simulink model "simulink_scheme_task2"  (R2023b)
settings: Solver=ode4  StartTime=0.0  StopTime=simulationParameters.T_sim  FixedStep=simulationParameters.T_integration  RelTol=1e-3
values from neighbouring files (symbols this model uses):
  patientParameters = loadPatientParameter(patientID)    [main_task_2.m]
  simulationParameters = loadSimulationParameter    [main_task_2.m]
settings Model: Creator=william  LastModifiedBy=william
settings DataIOCC: ReturnWorkspaceOutputs=off
settings ConfigComp: CovBoundaryAbsTol=1.0e-5

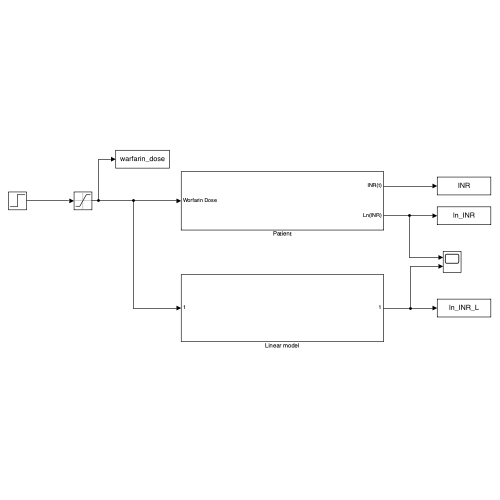
[thumbnail: Simulink's stored preview of the top-level diagram]
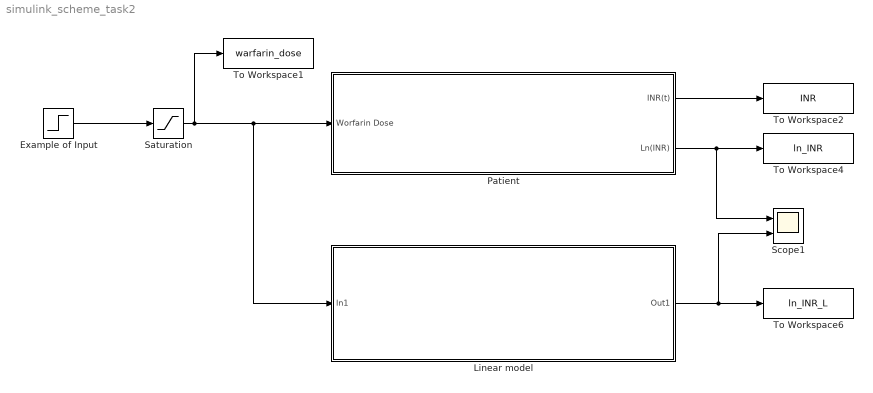
== system simulink_scheme_task2 ==
  Example of Input : Step  Time=48  After=4  SampleTime=simulationParameters.Ts
  Linear model : Subsystem
  Patient : Subsystem
  Saturation : Saturate  UpperLimit=simulationParameters.u_max  LowerLimit=simulationParameters.u_min
  Scope1 : Scope  NumInputPorts=2
  To Workspace1 : ToWorkspace  VariableName=warfarin_dose  SaveFormat=Structure With Time  SampleTime=-1
  To Workspace2 : ToWorkspace  VariableName=INR  SaveFormat=Structure With Time  SampleTime=-1
  To Workspace4 : ToWorkspace  VariableName=ln_INR  SaveFormat=Structure With Time  SampleTime=-1
  To Workspace6 : ToWorkspace  VariableName=ln_INR_L  SaveFormat=Structure With Time  SampleTime=-1
  wires:
  Saturation/1 -> Linear model/1(In1), Patient/1(Worfarin Dose), To Workspace1/1
  Patient/1(INR(t)) -> To Workspace2/1
  Patient/2(Ln(INR)) -> To Workspace4/1, Scope1/1
  Linear model/1(Out1) -> To Workspace6/1, Scope1/2
  Example of Input/1 -> Saturation/1

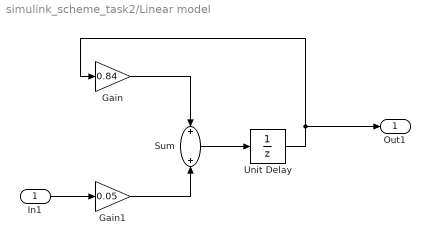
== system simulink_scheme_task2/Linear model ==
  In1 : Inport
  Gain : Gain  Gain=0.84
  Gain1 : Gain  Gain=0.05
  Sum : Sum
  Unit Delay : UnitDelay  SampleTime=simulationParameters.Ts
  Out1 : Outport
  wires:
  In1/1 -> Gain1/1
  Gain1/1 -> Sum/2
  Unit Delay/1 -> Gain/1, Out1/1
  Gain/1 -> Sum/1
  Sum/1 -> Unit Delay/1

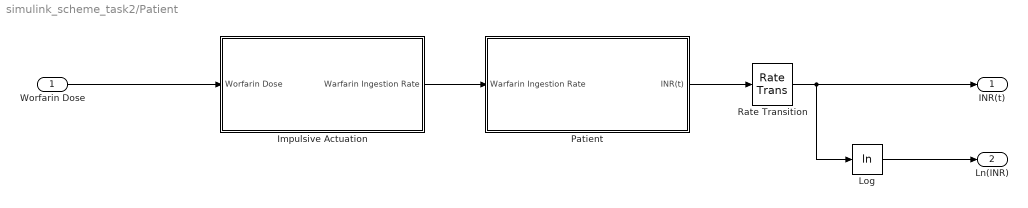
== system simulink_scheme_task2/Patient ==
  Worfarin Dose : Inport
  Impulsive Actuation : Subsystem
  Log : Math  Operator=log
  Patient : Subsystem
  Rate Transition : RateTransition  InitialCondition=patientParameters.BASE  OutPortSampleTime=simulationParameters.Ts
  INR(t) : Outport
  Ln(INR) : Outport  Port=2
  wires:
  Rate Transition/1 -> INR(t)/1, Log/1
  Worfarin Dose/1 -> Impulsive Actuation/1(Worfarin Dose)
  Impulsive Actuation/1(Warfarin Ingestion Rate) -> Patient/1("Warfarin Ingestion Rate ")
  Patient/1(INR(t)) -> Rate Transition/1
  Log/1 -> Ln(INR)/1

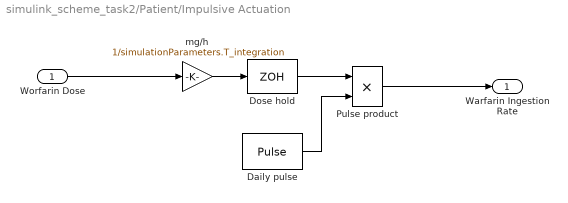
== system simulink_scheme_task2/Patient/Impulsive Actuation ==
  Worfarin Dose : Inport
  Daily pulse : DiscretePulseGenerator  Period=simulationParameters.Ts/simulationParameters.T_integration  SampleTime=simulationParameters.T_integration
  Dose hold : ZeroOrderHold  SampleTime=simulationParameters.T_integration
  Pulse product : Product  Inputs=**
  mg/h : Gain  Gain=1/simulationParameters.T_integration
  Warfarin Ingestion Rate : Outport
  wires:
  Worfarin Dose/1 -> mg/h/1
  mg/h/1 -> Dose hold/1
  Dose hold/1 -> Pulse product/1
  Daily pulse/1 -> Pulse product/2
  Pulse product/1 -> Warfarin Ingestion Rate/1

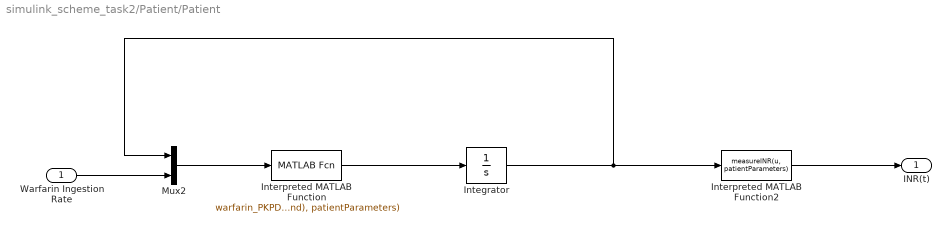
== system simulink_scheme_task2/Patient/Patient ==
  "Warfarin Ingestion Rate " : Inport
  Integrator : Integrator  InitialCondition=[patientParameters.x0,patientParameters.appearance.x0]
  Interpreted MATLAB Function : MATLABFcn  MATLABFcn=warfarin_PKPD_model(u(1:end-1), u(end), patientParameters)  OutputDimensions=8
  Interpreted MATLAB Function2 : MATLABFcn  MATLABFcn=measureINR(u, patientParameters)
  Mux2 : Mux  Inputs=2
  INR(t) : Outport
  wires:
  Interpreted MATLAB Function/1 -> Integrator/1
  Interpreted MATLAB Function2/1 -> INR(t)/1
  Integrator/1 -> Mux2/1, Interpreted MATLAB Function2/1
  Mux2/1 -> Interpreted MATLAB Function/1
  "Warfarin Ingestion Rate "/1 -> Mux2/2
